simulink model "MCU_Sensing"  (R2024a)
settings: Solver=VariableStepAuto  StartTime=0.0  StopTime=10.0  RelTol=1e-3
libraries: fl_lib x11, nesl_utility x3, ee_lib x1
settings Model: Creator=g_lautur  LastModifiedBy=g_lautur

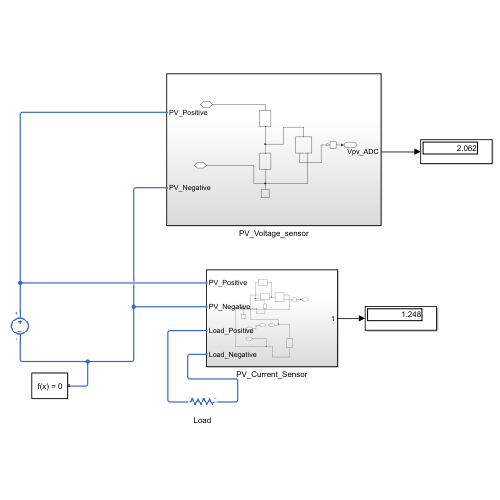
[thumbnail: Simulink's stored preview of the top-level diagram]
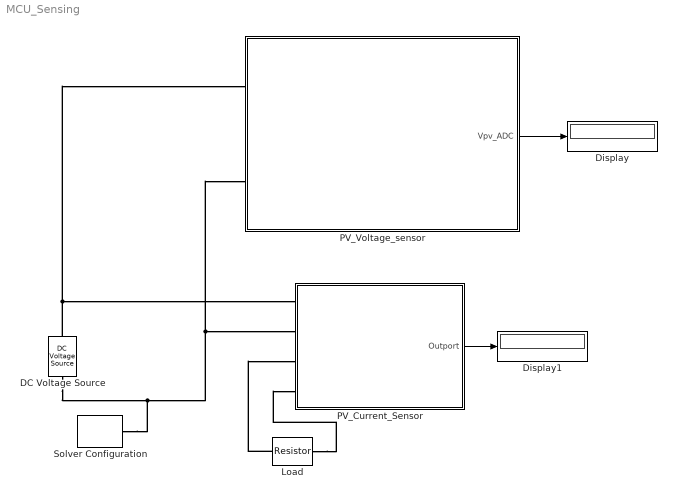
== system MCU_Sensing ==
  DC Voltage Source : ee_lib/Additional Components/SPICE Sources/DC Voltage Source  DC=33 V
  Display : Display
  Display1 : Display
  Load : fl_lib/Electrical/Electrical Elements/Resistor  R=3.3 Ohm  i_specify=off  i_priority=None  i=0 A  i_nominal_specify=off  i_nominal_value=1  i_nominal_unit=A  v_specify=off  v_priority=None  v=0 V  v_nominal_specify=off  v_nominal_value=1  v_nominal_unit=V
  PV_Current_Sensor : Subsystem
  PV_Voltage_sensor : Subsystem
  Solver Configuration : nesl_utility/Solver Configuration  PhysicalDomain=network_engine_domain  SubClassName=solver  LeftPortType=input  RightPortType=generic  Tones=[]  Harmonics=[]  SimulateNoise=off  Profile=off  UseLocalSampling=off  EnableSwitchedLinearOptims=on  FrequencyDomain=off  UseCCode=off  RelTol=0.001  AbsTol=0.001  MinStep=1e-09  ToWorkspace=off  RevertToSquareIcSolve=off  NumHomotopyIterations=100  PhasorMode=off  PhasorModeNumHarmonics=1  ConsistencySolver=NEWTON_XTOL_AFTER_FTOL  IndexReductionMethod=DerivativeReplacement  DoDC=off  ResidualTolerance=1e-09  ConsistencyTolSource=GLOBAL  ConsistencyAbsTol=0.001  ConsistencyRelTol=0.001  ConsistencyTolFactor=0.001  UseLocalSolver=off  LocalSolverChoice=NE_BACKWARD_EULER_ADVANCER  ResolveIndetEquations=on  FunctionEvalNumThread=1  LocalSolverSampleTime=0.001  DoFixedCost=off  MaxNonlinIter=3  MaxModeIter=2  ComputeImpulses=off  ImpulseIterations=2  LinearAlgebra=auto  LinearAlgebraNumThread=0  EquationFormulation=NE_TIME_EF  DelaysMemoryBudget=1024  AutomaticFiltering=on  FilteringTimeConstant=0.001  PartitionStorageMethod=AS_NEEDED  PartitionMemoryBudget=1024  PartitionMethod=ROBUST  MultibodyUseLocalSolver=off  MultibodyLocalSolverChoice=ODE1  MultibodyLocalSolverSampleTime=0.001
  wires:
  PV_Voltage_sensor/1(Vpv_ADC) -> Display/1
  PV_Current_Sensor/1(Outport) -> Display1/1
  connections:
  DC Voltage Source/LConn1 -- PV_Current_Sensor/LConn1 -- PV_Voltage_sensor/LConn1
  DC Voltage Source/RConn1 -- Solver Configuration/RConn1 -- PV_Current_Sensor/LConn2 -- PV_Voltage_sensor/LConn2
  Load/LConn1 -- PV_Current_Sensor/LConn3
  Load/RConn1 -- PV_Current_Sensor/LConn4

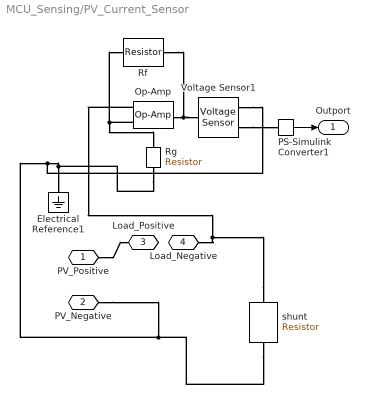
== system MCU_Sensing/PV_Current_Sensor ==
  Electrical Reference1 : fl_lib/Electrical/Electrical Elements/Electrical Reference
  Op-Amp : fl_lib/Electrical/Electrical Elements/Op-Amp  outI_specify=off  outI_priority=None  outI=0 A  outI_nominal_specify=off  outI_nominal_value=1  outI_nominal_unit=A
  PS-Simulink Converter1 : nesl_utility/PS-Simulink Converter  PhysicalDomain=network_engine_domain  SubClassName=ps_output  LeftPortType=input  RightPortType=output  PseudoPeriodic=off  Frequencies=[]  VectorFormat=inherit  Unit=inherit  AffineConversion=off
  Rf : fl_lib/Electrical/Electrical Elements/Resistor  R=240 kOhm  i_specify=off  i_priority=None  i=0 A  i_nominal_specify=off  i_nominal_value=1  i_nominal_unit=A  v_specify=off  v_priority=None  v=0 V  v_nominal_specify=off  v_nominal_value=1  v_nominal_unit=V
  Rg : fl_lib/Electrical/Electrical Elements/Resistor  R=10 kOhm  i_specify=off  i_priority=None  i=0 A  i_nominal_specify=off  i_nominal_value=1  i_nominal_unit=A  v_specify=off  v_priority=None  v=0 V  v_nominal_specify=off  v_nominal_value=1  v_nominal_unit=V
  Voltage Sensor1 : fl_lib/Electrical/Electrical Sensors/Voltage Sensor
  shunt : fl_lib/Electrical/Electrical Elements/Resistor  R=0.005 Ohm  i_specify=off  i_priority=None  i=0 A  i_nominal_specify=off  i_nominal_value=1  i_nominal_unit=A  v_specify=off  v_priority=None  v=0 V  v_nominal_specify=off  v_nominal_value=1  v_nominal_unit=V
  PV_Positive : PMIOPort  Side=Left
  PV_Negative : PMIOPort  Port=2  Side=Left
  Load_Positive : PMIOPort  Port=3  Side=Left
  Load_Negative : PMIOPort  Port=4  Side=Left
  Outport : Outport
  wires:
  PS-Simulink Converter1/1 -> Outport/1
  connections:
  Op-Amp/RConn1 -- Rf/RConn1 -- Voltage Sensor1/LConn1
  PV_Negative/RConn1 -- shunt/RConn1 -- Voltage Sensor1/RConn2 -- Rg/RConn1 -- Electrical Reference1/LConn1
  Op-Amp/LConn2 -- Rf/LConn1 -- Rg/LConn1
  Voltage Sensor1/RConn1 -- PS-Simulink Converter1/LConn1
  shunt/LConn1 -- Load_Negative/RConn1 -- Op-Amp/LConn1
  PV_Positive/RConn1 -- Load_Positive/RConn1

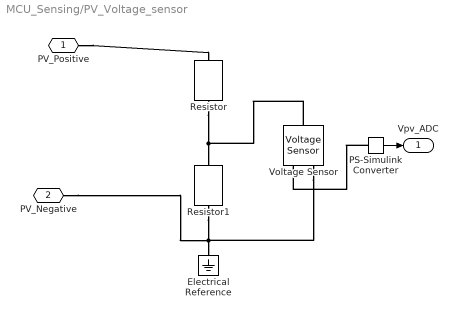
== system MCU_Sensing/PV_Voltage_sensor ==
  Electrical Reference : fl_lib/Electrical/Electrical Elements/Electrical Reference
  PS-Simulink Converter : nesl_utility/PS-Simulink Converter  PhysicalDomain=network_engine_domain  SubClassName=ps_output  LeftPortType=input  RightPortType=output  PseudoPeriodic=off  Frequencies=[]  VectorFormat=inherit  Unit=inherit  AffineConversion=off
  Resistor : fl_lib/Electrical/Electrical Elements/Resistor  R=150 kOhm  i_specify=off  i_priority=None  i=0 A  i_nominal_specify=off  i_nominal_value=1  i_nominal_unit=A  v_specify=off  v_priority=None  v=0 V  v_nominal_specify=off  v_nominal_value=1  v_nominal_unit=V
  Resistor1 : fl_lib/Electrical/Electrical Elements/Resistor  R=10 kOhm  i_specify=off  i_priority=None  i=0 A  i_nominal_specify=off  i_nominal_value=1  i_nominal_unit=A  v_specify=off  v_priority=None  v=0 V  v_nominal_specify=off  v_nominal_value=1  v_nominal_unit=V
  Voltage Sensor : fl_lib/Electrical/Electrical Sensors/Voltage Sensor
  PV_Positive : PMIOPort  Side=Left
  PV_Negative : PMIOPort  Port=2  Side=Left
  Vpv_ADC : Outport
  wires:
  PS-Simulink Converter/1 -> Vpv_ADC/1
  connections:
  PS-Simulink Converter/LConn1 -- Voltage Sensor/RConn1
  Resistor1/RConn1 -- PV_Negative/RConn1 -- Voltage Sensor/RConn2 -- Electrical Reference/LConn1
  Resistor/RConn1 -- Voltage Sensor/LConn1 -- Resistor1/LConn1
  PV_Positive/RConn1 -- Resistor/LConn1
